simulink model "LabB_TuneTheGyro"  (R2020a)
settings: Solver=FixedStepDiscrete  StartTime=0.0  StopTime=inf  FixedStep=fSamplingPeriod  RelTol=1e-3  EnableMultiTasking=on
libraries: simulink x1
settings Model: FPTRunName=FPA_Reference  SimulationMode=external  ExtModeTrigDuration=2  Creator=Alec  LastModifiedBy=khaatt
settings DataIOCC: SaveFormat=Array  SaveOutput=off  SignalLogging=off  DSMLogging=off  SaveTime=off  ReturnWorkspaceOutputs=off
settings OptimizationCC: PassReuseOutputArgsAs=Individual arguments  ExpressionDepthLimit=2147483647  MaxStackSize=64  EfficientTunableParamExpr=on
settings DebuggingCC: UnderspecifiedInitializationDetection=Classic  MergeDetectMultiDrivingBlocksExec=none  ParameterTunabilityLossMsg=error  StateNameClashWarn=warning  SFUnexpectedBacktrackingDiag=warning  SFNoUnconditionalDefaultTransitionDiag=warning  SFExecutionAtInitializationDiag=none  ArithmeticOperatorsInVariantConditions=warning
settings HardwareCC: ProdBitPerInt=16  ProdBitPerPointer=16  ProdBitPerSizeT=16  ProdBitPerPtrDiffT=16  ProdLargestAtomicFloat=None  ProdWordSize=8  ProdHWDeviceType=Atmel->AVR
settings ModelReferenceCC: PropagateSignalLabelsOutOfModel=off
settings SFSimCC: SimUseLocalCustomCode=off  MATLABDynamicMemAlloc=off  CustomCodeUndefinedFunction=UseInterfaceOnly
settings RTWCC: SystemTargetFile=ert.tlc  HardwareBoard=Arduino Mega 2560  TLCOptions=-aInlineSetEventsForThisBaseRateFcn=TLC_FALSE -aSuppressMultiTaskScheduler=TLC_FALSE -aRateBasedStepFcn=1  TemplateMakefile=ert_default_tmf  GenerateReport=on  RTWVerbose=off  RTWUseLocalCustomCode=off  Toolchain=Arduino AVR  BuildConfiguration=Faster Runs  IncludeHyperlinkInReport=on  LaunchReport=on  GenerateTraceInfo=on  GenerateTraceReport=on  GenerateTraceReportSl=on  GenerateTraceReportSf=on  GenerateTraceReportEml=on
settings CodeAppCC: ForceParamTrailComments=on  IgnoreCustomStorageClasses=off  OperatorAnnotations=on  SimulinkDataObjDesc=on  SFDataObjDesc=on  MATLABFcnDesc=on  CustomSymbolStrType=$N$R$M  InsertBlockDesc=on  StateflowObjectComments=on  MATLABSourceComments=on  InternalIdentifier=Classic
settings ERTTargetCC: SupportContinuousTime=on  SupportVariableSizeSignals=on
settings ConfigComp: CovMetricSettings=dw  CovHtmlReporting=on  CovSaveCumulativeToWorkspaceVar=on  CovSaveSingleToWorkspaceVar=on  CovExternalEMLEnable=off

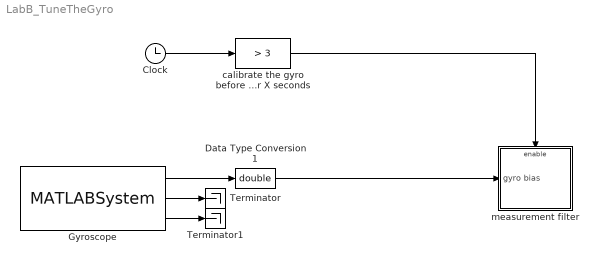
== system LabB_TuneTheGyro ==
  Clock : Clock
  Data Type Conversion1 : DataTypeConversion  OutDataTypeStr=double
  Gyroscope : MATLABSystem  System=soMPU6050Gyro  DLPFmode=0
      mask Type: soMPU6050Gyro
      mask Display:
      | disp('soMPU6050Gyro');
      | port_label('output',1,'xvel');
      | port_label('output',2,'yvel');
      | port_label('output',3,'zvel');
  Terminator : Terminator
  Terminator1 : Terminator
  "calibrate the gyro before X seconds, start controlling after X seconds" : simulink/Logic and Bit Operations/Compare To Constant  relop=>  const=3  OutDataTypeStr=boolean
  measurement filter : Subsystem
  wires:
  Clock/1 -> "calibrate the gyro before X seconds, start controlling after X seconds"/1
  "calibrate the gyro before X seconds, start controlling after X seconds"/1 -> measurement filter/Enable
  Data Type Conversion1/1 -> measurement filter/1(gyro bias)
  Gyroscope/1 -> Data Type Conversion1/1
  Gyroscope/2 -> Terminator/1
  Gyroscope/3 -> Terminator1/1

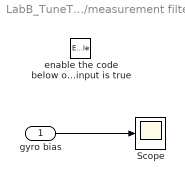
== system LabB_TuneTheGyro/measurement filter ==
  gyro bias : Inport
  "enable the code below only when the external boolean input is true " : EnablePort
  Scope : Scope
  wires:
  gyro bias/1 -> Scope/1
